simulink model "encelado"  (R2022b)
settings: Solver=ode4  StartTime=0.0  StopTime=500  FixedStep=0.01  RelTol=1e-3
values from neighbouring files (symbols this model uses):
  ba0 = 1e-3*randn(3,1)    [enceladus.m]
  bg0 = deg2rad(10/3600)*randn(3,1)    [enceladus.m]
  dp_in = [-5;40;0]    [enceladus.m]
  dt_alt = 0.1    [enceladus.m]
  dt_cam = 1    [enceladus.m]
  dt_imu = 0.02    [enceladus.m]
  Frcs = 22    [enceladus.m]
  g0 = 9.80665    [enceladus.m]
  Gam = 0.005    [enceladus.m]
  hth = 0.5    [enceladus.m]
  Isp = 300    [enceladus.m]
  Isp_rcs = 290    [enceladus.m]
  k_c = 0.01    [enceladus.m]
  k_h = 0.005    [enceladus.m]
  kC = 1    [enceladus.m]
  kd = 2*zeta*wn*J    [enceladus.m]
  Km = 5    [enceladus.m]
  kp = 2*J*wn^2    [enceladus.m]
  kS = 1    [enceladus.m]
  kw = 1    [enceladus.m]
  L = (P-r_sito')*E    [enceladus.m]
  m_in = 1000    [enceladus.m]
  mu = 7.21e9    (= 7210000000)    [enceladus.m]
  n = sqrt(muS/a^3)    [enceladus.m]
  N_alt = round(dt_alt/dt_imu)    [enceladus.m]
  N_cam = round(dt_cam/dt_imu)    [enceladus.m]
  N_st = round(dt_st/dt_imu)    [enceladus.m]
  P0 = diag([sigma_p0^2*ones(1,3),sigma_v0^2*ones(1,3),sigma_b0^2*ones(1,3)])    [enceladus.m]
  p_in = (R+h0)*uf    [enceladus.m]
  Pa0 = blkdiag(sigma_th0^2*eye(3),sigma_bg0^2*eye(3))    [enceladus.m]
  pf = (R-0.5)*u_f    [enceladus.m]
  q_in = [1 0 0 0]'    [enceladus.m]
  R = 252.1e3    (= 252100)    [enceladus.m]
  r_off = [0;0;0]    [enceladus.m]
  sigma_a = 5e-4    (= 0.0005)    [enceladus.m]
  sigma_ba = 1e-6    (= 1e-06)    [enceladus.m]
  sigma_c0 = 0.5    [enceladus.m]
  sigma_h0 = 0.2    [enceladus.m]
  sigma_st = 5e-5    (= 5e-05)    [enceladus.m]
  sigma_u = 1e-8    (= 1e-08)    [enceladus.m]
  sigma_v = 1e-5    (= 1e-05)    [enceladus.m]
  taumax_rcs = 2*Frcs*L    (= 26.4)    [enceladus.m]
  tgo_min = 10    [enceladus.m]
  Tm = 0.4    [enceladus.m]
  Uoff = 0.05    [enceladus.m]
  Uon = 0.2    [enceladus.m]
  vf = [0;0;0]    [enceladus.m]
  w_in = [0 0 0]'    [enceladus.m]
  x0_hat = [p_in+sigma_p0*randn(3,1);dp_in+sigma_v0*randn(3,1);zeros(3,1)]    [enceladus.m]
  xa0 = [q_hat0;zeros(3,1)]    [enceladus.m]
undefined symbols (not defined in the file or in its folder): h_rw_in, hmax_rw, tau_rcs, taumax_rw
libraries: simulink x1
settings Model: Creator=lorenzocipolla  LastModifiedBy=lorenzocipolla

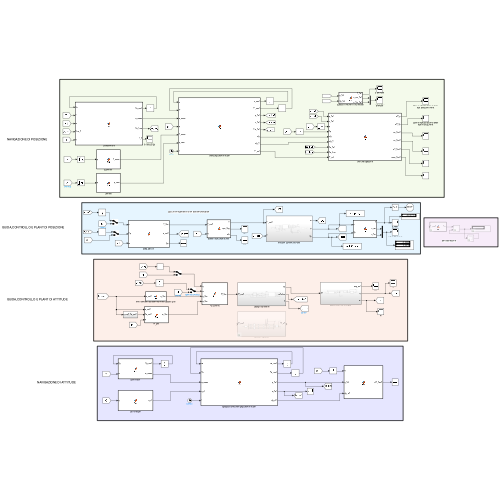
[thumbnail: Simulink's stored preview of the top-level diagram]
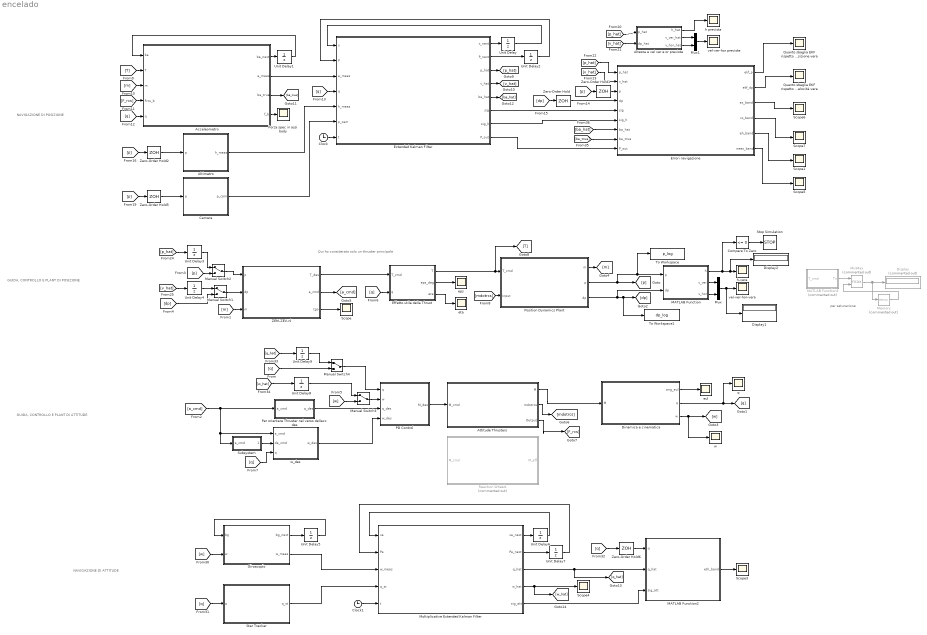
== system encelado ==
  note: NAVIGAZIONE DI POSIZIONE
  note: Qui ho considerato solo un thruster principale
  note: per saturazione
  note: GUIDA, CONTROLLO E PLANT DI POSIZIONE
  note: GUIDA, CONTROLLO E PLANT DI ATTITUDE
  note: NAVIGAZIONE DI ATTITUDE
  Acceleometro : MATLAB Function  TreatAsAtomicUnit=on
  Altezza e vel ver e or previste : MATLAB Function  TreatAsAtomicUnit=on
  Altimetro : MATLAB Function  TreatAsAtomicUnit=on
  Attitude Thrusters : Subsystem
  Camera : MATLAB Function  TreatAsAtomicUnit=on
  Clock : Clock
  Clock1 : Clock
  Compare To Zero : simulink/Logic and Bit Operations/Compare To Zero  relop=<=  OutDataTypeStr=boolean
  Dinamica e cinematica : Subsystem
  Display : Display  Commented=on
  Display1 : Display
  Display2 : Display
  Effetto utile della Thrust : MATLAB Function  TreatAsAtomicUnit=on
  Errori navigazione : MATLAB Function  TreatAsAtomicUnit=on
  Extended Kalman Filter : MATLAB Function  TreatAsAtomicUnit=on
  Forza spec in assi body : Scope
  Giroscopio : MATLAB Function  TreatAsAtomicUnit=on
  MATLAB Function : MATLAB Function  TreatAsAtomicUnit=on
  MATLAB Function2 : MATLAB Function  TreatAsAtomicUnit=on
  MATLAB Function3 : MATLAB Function  Commented=on  TreatAsAtomicUnit=on
  Manual Switch{1..4} (4 alike) : ManualSwitch
  Memory : Memory  Commented=on
  MinMax : MinMax  Commented=on  Function=max  Inputs=2
  Moltiplicative Extended Kalman Filter : MATLAB Function  TreatAsAtomicUnit=on
  Mux : Mux  Inputs=2
  Mux1 : Mux  Inputs=2
  PD Control : MATLAB Function  TreatAsAtomicUnit=on
  Per orientare Thruster nel verso dellacc des : MATLAB Function  TreatAsAtomicUnit=on
  Position Dynamics Plant : Subsystem
  Quanto sbaglia EKF rispetto alla posizione vera : Scope
  Quanto sbaglia EKF rispetto alla velocità vera : Scope
  Reaction Wheels : Subsystem  Commented=on
  Scope{,1,3..7} (7 alike) : Scope
  Star Tracker : MATLAB Function  TreatAsAtomicUnit=on
  Stop Simulation : Stop
  Subsystem : Subsystem
  To Workspace : ToWorkspace  VariableName=p_log  SampleTime=-1
  To Workspace1 : ToWorkspace  VariableName=dp_log  SampleTime=-1
  Unit Delay : UnitDelay  InitialCondition=x0_hat  SampleTime=dt_imu  HasFrameUpgradeWarning=on
  Unit Delay1 : UnitDelay  InitialCondition=ba0  SampleTime=dt_imu  HasFrameUpgradeWarning=on
  Unit Delay2 : UnitDelay  InitialCondition=P0  SampleTime=dt_imu  HasFrameUpgradeWarning=on
  Unit Delay3 : UnitDelay  InitialCondition=x0_hat(1:3)  SampleTime=dt_imu  HasFrameUpgradeWarning=on
  Unit Delay4 : UnitDelay  InitialCondition=x0_hat(4:6)  SampleTime=dt_imu  HasFrameUpgradeWarning=on
  Unit Delay5 : UnitDelay  InitialCondition=bg0  SampleTime=dt_imu  HasFrameUpgradeWarning=on
  Unit Delay6 : UnitDelay  InitialCondition=xa0  SampleTime=dt_imu  HasFrameUpgradeWarning=on
  Unit Delay7 : UnitDelay  InitialCondition=Pa0  SampleTime=dt_imu  HasFrameUpgradeWarning=on
  Unit Delay8 : UnitDelay  InitialCondition=xa0(5:7)  SampleTime=dt_imu  HasFrameUpgradeWarning=on
  Unit Delay9 : UnitDelay  InitialCondition=xa0(1:4)  SampleTime=dt_imu  HasFrameUpgradeWarning=on
  ZEM-ZEV-nl : MATLAB Function  TreatAsAtomicUnit=on
  Zero-Order Hold : ZeroOrderHold  SampleTime=dt_imu
  Zero-Order Hold1 : ZeroOrderHold  SampleTime=dt_imu
  Zero-Order Hold2 : ZeroOrderHold  SampleTime=dt_alt
  Zero-Order Hold5 : ZeroOrderHold  SampleTime=dt_cam
  Zero-Order Hold6 : ZeroOrderHold  SampleTime=dt_imu
  eps : Scope
  eta : Scope
  eul : Scope
  h prevista : Scope
  h-vera : Scope
  q : Scope
  vel-ver-hor previste : Scope
  vel-ver-hor-vera : Scope
  w : Scope
  w_des : MATLAB Function  TreatAsAtomicUnit=on
  wires:
  MinMax/1 -> Memory/1, Display/1
  Memory/1 -> MinMax/2
  MATLAB Function3/1(Tn) -> MinMax/1
  Dinamica e cinematica/1(ang_eul) -> eul/1
  Dinamica e cinematica/2(q) -> q/1, [q]
  Dinamica e cinematica/3(w) -> [w], w/1
  Position Dynamics Plant/2(p) -> To Workspace/1, MATLAB Function/1(p), [p]
  Position Dynamics Plant/3(dp) -> MATLAB Function/2(dp), To Workspace1/1, [dp]
  Position Dynamics Plant/1(m) -> [m]
  MATLAB Function/1(h) -> Display2/1, h-vera/1, Compare To Zero/1
  MATLAB Function/2(v_ver) -> Mux/1
  MATLAB Function/3(v_hor) -> Mux/2
  Mux/1 -> vel-ver-hor-vera/1, Display1/1
  [m] -> ZEM-ZEV-nl/3(m)
  ZEM-ZEV-nl/2(a_cmd) -> [a_cmd]
  [q] -> Effetto utile della Thrust/2(q)
  Effetto utile della Thrust/1(T) -> [T], Position Dynamics Plant/1(T_cmd)
  Effetto utile della Thrust/3(eta) -> eta/1
  Effetto utile della Thrust/2(eps_deg) -> eps/1
  ZEM-ZEV-nl/1(T_des) -> Effetto utile della Thrust/1(T_cmd)
  Compare To Zero/1 -> Stop Simulation/1
  ZEM-ZEV-nl/3(tgo) -> Scope/1
  Per orientare Thruster nel verso dellacc des/1(q_des) -> PD Control/3(q_des)
  w_des/1(w_des) -> PD Control/4(w_des)
  [a_cmd] -> Subsystem/1(a_cmd), w_des/1(a_cmd), Per orientare Thruster nel verso dellacc des/1(a_cmd)
  Subsystem/1(da_cmd) -> w_des/2(da_cmd)
  [q] -> w_des/3(q)
  PD Control/1(M_des) -> Attitude Thrusters/1(M_cmd)
  Attitude Thrusters/1(M) -> Dinamica e cinematica/1(M)
  [mdotrcs] -> Position Dynamics Plant/2(Input)
  Attitude Thrusters/2(mdotrcs) -> [mdotrcs]
  [T] -> Acceleometro/2(T)
  Attitude Thrusters/3(Output) -> [F_rcs]
  [F_rcs] -> Acceleometro/4(Frcs_b)
  [m] -> Acceleometro/3(m)
  [q] -> Acceleometro/5(q)
  Extended Kalman Filter/1(x_next) -> Unit Delay/1
  Unit Delay/1 -> Extended Kalman Filter/1(x)
  Acceleometro/1(ba_next) -> Unit Delay1/1
  Unit Delay1/1 -> Acceleometro/1(ba)
  Acceleometro/2(a_meas) -> Extended Kalman Filter/3(a_meas)
  [q] -> Extended Kalman Filter/4(q)
  Acceleometro/4(f_b) -> Forza spec in assi body/1
  Altezza e vel ver e or previste/3(v_hor_hat) -> Mux1/2
  Altezza e vel ver e or previste/2(v_ver_hat) -> Mux1/1
  Altezza e vel ver e or previste/1(h_hat) -> h prevista/1
  Mux1/1 -> vel-ver-hor previste/1
  Errori navigazione/1(ekf_p) -> Quanto sbaglia EKF rispetto alla posizione vera/1
  Errori navigazione/2(ekf_dp) -> Quanto sbaglia EKF rispetto alla velocità vera/1
  [p] -> Zero-Order Hold1/1
  Zero-Order Hold1/1 -> Errori navigazione/3(p)
  Zero-Order Hold/1 -> Errori navigazione/4(dp)
  [dp] -> Zero-Order Hold/1
  Errori navigazione/3(ex_band) -> Scope6/1
  Errori navigazione/4(vx_band) -> Scope7/1
  Extended Kalman Filter/2(P_next) -> Unit Delay2/1
  Unit Delay2/1 -> Extended Kalman Filter/2(P)
  Extended Kalman Filter/6(sig) -> Errori navigazione/5(sig)
  [p] -> Zero-Order Hold2/1
  Zero-Order Hold2/1 -> Altimetro/1(p)
  Clock/1 -> Extended Kalman Filter/7(t)
  Altimetro/1(h_meas) -> Extended Kalman Filter/5(h_meas)
  Extended Kalman Filter/7(sig_h) -> Errori navigazione/6(sig_h)
  Errori navigazione/5(eh_band) -> Scope1/1
  Camera/1(p_cam) -> Extended Kalman Filter/6(p_cam)
  [p] -> Zero-Order Hold5/1
  Zero-Order Hold5/1 -> Camera/1(p)
  Extended Kalman Filter/4(v_hat) -> [v_hat]
  Extended Kalman Filter/3(p_hat) -> [p_hat]
  [p_hat] -> Altezza e vel ver e or previste/1(p_hat)
  [v_hat] -> Altezza e vel ver e or previste/2(dp_hat)
  [p_hat] -> Errori navigazione/1(p_hat)
  [v_hat] -> Errori navigazione/2(v_hat)
  Acceleometro/3(ba_true) -> [ba_true]
  Extended Kalman Filter/5(ba_hat) -> [ba_hat]
  [p_hat] -> Unit Delay3/1
  [v_hat] -> Unit Delay4/1
  Manual Switch1/1 -> ZEM-ZEV-nl/2(dp)
  Manual Switch2/1 -> ZEM-ZEV-nl/1(p)
  [p] -> Manual Switch2/2
  Unit Delay3/1 -> Manual Switch2/1
  Unit Delay4/1 -> Manual Switch1/1
  [dp] -> Manual Switch1/2
  [w] -> Giroscopio/2(w)
  Giroscopio/1(bg_next) -> Unit Delay5/1
  Unit Delay5/1 -> Giroscopio/1(bg)
  [q] -> Star Tracker/1(q)
  Moltiplicative Extended Kalman Filter/1(xa_next) -> Unit Delay6/1
  Unit Delay6/1 -> Moltiplicative Extended Kalman Filter/1(xa)
  Giroscopio/2(w_meas) -> Moltiplicative Extended Kalman Filter/3(w_meas)
  Moltiplicative Extended Kalman Filter/3(q_hat) -> [q_hat], MATLAB Function2/2(q_hat)
  Moltiplicative Extended Kalman Filter/5(sig_att) -> MATLAB Function2/3(sig_att)
  MATLAB Function2/1(eth_band) -> Scope3/1
  Moltiplicative Extended Kalman Filter/2(Pa_next) -> Unit Delay7/1
  Unit Delay7/1 -> Moltiplicative Extended Kalman Filter/2(Pa)
  Star Tracker/1(q_st) -> Moltiplicative Extended Kalman Filter/4(q_st)
  Zero-Order Hold6/1 -> MATLAB Function2/1(q)
  [q] -> Zero-Order Hold6/1
  Clock1/1 -> Moltiplicative Extended Kalman Filter/5(t)
  Moltiplicative Extended Kalman Filter/4(w_hat) -> [w_hat], Scope4/1
  [q_hat] -> Unit Delay9/1
  [w_hat] -> Unit Delay8/1
  Manual Switch3/1 -> PD Control/2(w)
  [w] -> Manual Switch3/2
  Unit Delay8/1 -> Manual Switch3/1
  [q] -> Manual Switch4/2
  Unit Delay9/1 -> Manual Switch4/1
  Manual Switch4/1 -> PD Control/1(q)
  Errori navigazione/6(nees_band) -> Scope5/1
  [ba_true] -> Errori navigazione/8(ba_true)
  [ba_hat] -> Errori navigazione/7(ba_hat)
  Extended Kalman Filter/8(P_out) -> Errori navigazione/9(P_out)

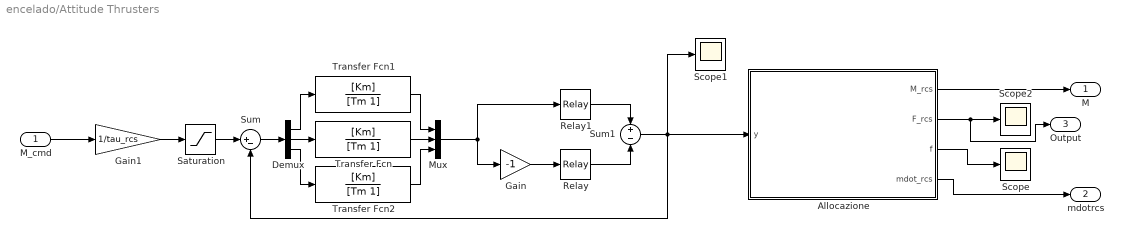
== system encelado/Attitude Thrusters ==
  M_cmd : Inport
  Allocazione : MATLAB Function  TreatAsAtomicUnit=on
  Demux : Demux  Outputs=3
  Gain : Gain  Gain=-1
  Gain1 : Gain  Gain=1/tau_rcs
  Mux : Mux  Inputs=3
  Relay : Relay  OnSwitchValue=Uon  OffSwitchValue=Uoff
  Relay1 : Relay  OnSwitchValue=Uon  OffSwitchValue=Uoff
  Saturation : Saturate  UpperLimit=taumax_rcs  LowerLimit=-taumax_rcs
  Scope : Scope
  Scope1 : Scope
  Scope2 : Scope
  Sum : Sum  Inputs=|+-
  Sum1 : Sum  Inputs=+|-
  Transfer Fcn : TransferFcn  Numerator=[Km]  Denominator=[Tm 1]
  Transfer Fcn1 : TransferFcn  Numerator=[Km]  Denominator=[Tm 1]
  Transfer Fcn2 : TransferFcn  Numerator=[Km]  Denominator=[Tm 1]
  M : Outport
  mdotrcs : Outport  Port=2
  Output : Outport  Port=3
  wires:
  Gain/1 -> Relay/1
  Sum1/1 -> Allocazione/1(y), Sum/2, Scope1/1
  Saturation/1 -> Sum/1
  Relay/1 -> Sum1/2
  Relay1/1 -> Sum1/1
  Gain1/1 -> Saturation/1
  Sum/1 -> Demux/1
  Demux/2 -> Transfer Fcn/1
  Transfer Fcn/1 -> Mux/2
  Demux/1 -> Transfer Fcn1/1
  Demux/3 -> Transfer Fcn2/1
  Transfer Fcn1/1 -> Mux/1
  Transfer Fcn2/1 -> Mux/3
  Mux/1 -> Gain/1, Relay1/1
  Allocazione/4(mdot_rcs) -> mdotrcs/1
  Allocazione/2(F_rcs) -> Output/1, Scope2/1
  Allocazione/3(f) -> Scope/1
  Allocazione/1(M_rcs) -> M/1
  M_cmd/1 -> Gain1/1

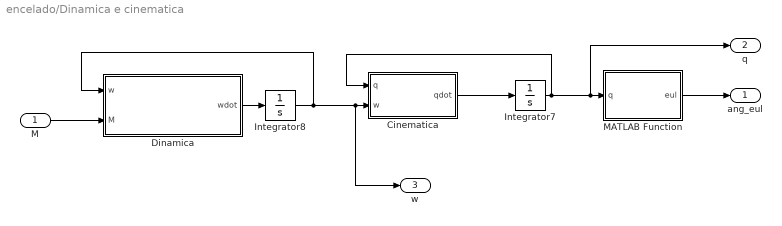
== system encelado/Dinamica e cinematica ==
  M : Inport
  Cinematica : MATLAB Function  TreatAsAtomicUnit=on
  Dinamica : MATLAB Function  TreatAsAtomicUnit=on
  Integrator7 : Integrator  InitialCondition=q_in
  Integrator8 : Integrator  InitialCondition=w_in
  MATLAB Function : MATLAB Function  TreatAsAtomicUnit=on
  ang_eul : Outport
  q : Outport  Port=2
  w : Outport  Port=3
  wires:
  Integrator7/1 -> q/1, MATLAB Function/1(q), Cinematica/1(q)
  Cinematica/1(qdot) -> Integrator7/1
  Dinamica/1(wdot) -> Integrator8/1
  MATLAB Function/1(eul) -> ang_eul/1
  Integrator8/1 -> Dinamica/1(w), w/1, Cinematica/2(w)
  M/1 -> Dinamica/2(M)

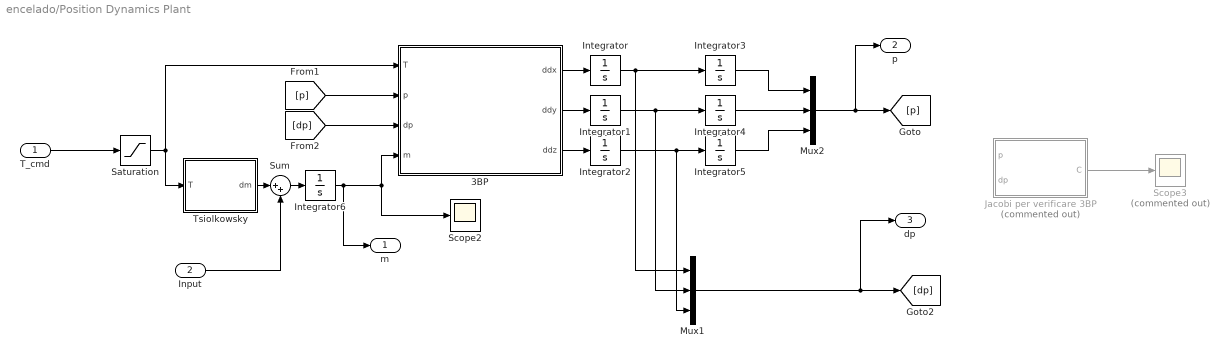
== system encelado/Position Dynamics Plant ==
  T_cmd : Inport
  Input : Inport  Port=2
  3BP : MATLAB Function  TreatAsAtomicUnit=on
  Integrator : Integrator  InitialCondition=dp_in(1)
  Integrator1 : Integrator  InitialCondition=dp_in(2)
  Integrator2 : Integrator  InitialCondition=dp_in(3)
  Integrator3 : Integrator  InitialCondition=p_in(1)
  Integrator4 : Integrator  InitialCondition=p_in(2)
  Integrator5 : Integrator  InitialCondition=p_in(3)
  Integrator6 : Integrator  InitialCondition=m_in
  Jacobi per verificare 3BP : MATLAB Function  Commented=on  TreatAsAtomicUnit=on
  Mux1 : Mux  Inputs=3
  Mux2 : Mux  Inputs=3
  Saturation : Saturate  UpperLimit=700  LowerLimit=-700
  Scope2 : Scope
  Scope3 : Scope  Commented=on
  Sum : Sum  Inputs=|++
  Tsiolkowsky : MATLAB Function  TreatAsAtomicUnit=on
  m : Outport
  p : Outport  Port=2
  dp : Outport  Port=3
  wires:
  3BP/3(ddz) -> Integrator2/1
  Integrator4/1 -> Mux2/2
  Mux1/1 -> dp/1, [dp]
  3BP/1(ddx) -> Integrator/1
  Integrator5/1 -> Mux2/3
  Mux2/1 -> p/1, [p]
  Integrator6/1 -> Scope2/1, 3BP/4(m), m/1
  Integrator2/1 -> Integrator5/1, Mux1/3
  Integrator/1 -> Mux1/1, Integrator3/1
  Saturation/1 -> 3BP/1(T), Tsiolkowsky/1(T)
  Integrator3/1 -> Mux2/1
  Integrator1/1 -> Mux1/2, Integrator4/1
  T_cmd/1 -> Saturation/1
  3BP/2(ddy) -> Integrator1/1
  [p] -> 3BP/2(p)
  [dp] -> 3BP/3(dp)
  Jacobi per verificare 3BP/1(C) -> Scope3/1
  Tsiolkowsky/1(dm) -> Sum/1
  Sum/1 -> Integrator6/1
  Input/1 -> Sum/2

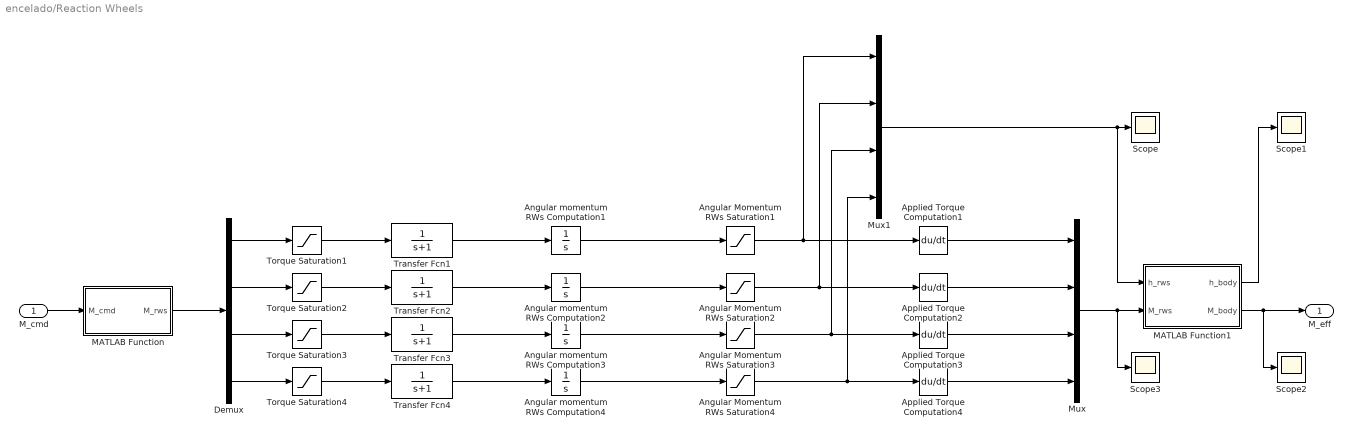
== system encelado/Reaction Wheels ==
  M_cmd : Inport
  Angular Momentum RWs Saturation{1..4} (4 alike) : Saturate  UpperLimit=hmax_rw  LowerLimit=-hmax_rw
  Angular momentum RWs Computation1 : Integrator  InitialCondition=h_rw_in(1)
  Angular momentum RWs Computation2 : Integrator  InitialCondition=h_rw_in(2)
  Angular momentum RWs Computation3 : Integrator  InitialCondition=h_rw_in(3)
  Angular momentum RWs Computation4 : Integrator  InitialCondition=h_rw_in(4)
  Applied Torque Computation{1..4} (4 alike) : Derivative  CoefficientInTFapproximation=0.01
  Demux : Demux
  MATLAB Function : MATLAB Function  TreatAsAtomicUnit=on
  MATLAB Function1 : MATLAB Function  TreatAsAtomicUnit=on
  Mux : Mux
  Mux1 : Mux
  Scope{,1..3} (4 alike) : Scope
  Torque Saturation{1..4} (4 alike) : Saturate  UpperLimit=taumax_rw  LowerLimit=-taumax_rw
  Transfer Fcn{1..4} (4 alike) : TransferFcn  Denominator=[1 1]
  M_eff : Outport
  wires:
  M_cmd/1 -> MATLAB Function/1(M_cmd)
  MATLAB Function/1(M_rws) -> Demux/1
  Torque Saturation1/1 -> Transfer Fcn1/1
  Transfer Fcn2/1 -> Angular momentum RWs Computation2/1
  Demux/2 -> Torque Saturation2/1
  Angular Momentum RWs Saturation3/1 -> Mux1/3, Applied Torque Computation3/1
  Torque Saturation4/1 -> Transfer Fcn4/1
  Torque Saturation2/1 -> Transfer Fcn2/1
  Angular momentum RWs Computation2/1 -> Angular Momentum RWs Saturation2/1
  Transfer Fcn4/1 -> Angular momentum RWs Computation4/1
  Angular Momentum RWs Saturation1/1 -> Mux1/1, Applied Torque Computation1/1
  Applied Torque Computation4/1 -> Mux/4
  Angular momentum RWs Computation3/1 -> Angular Momentum RWs Saturation3/1
  Torque Saturation3/1 -> Transfer Fcn3/1
  Angular Momentum RWs Saturation2/1 -> Mux1/2, Applied Torque Computation2/1
  Applied Torque Computation3/1 -> Mux/3
  Angular momentum RWs Computation4/1 -> Angular Momentum RWs Saturation4/1
  Demux/1 -> Torque Saturation1/1
  Applied Torque Computation2/1 -> Mux/2
  Applied Torque Computation1/1 -> Mux/1
  Transfer Fcn3/1 -> Angular momentum RWs Computation3/1
  Angular momentum RWs Computation1/1 -> Angular Momentum RWs Saturation1/1
  Demux/3 -> Torque Saturation3/1
  Transfer Fcn1/1 -> Angular momentum RWs Computation1/1
  Angular Momentum RWs Saturation4/1 -> Mux1/4, Applied Torque Computation4/1
  Demux/4 -> Torque Saturation4/1
  MATLAB Function1/2(M_body) -> Scope2/1, M_eff/1
  Mux/1 -> Scope3/1, MATLAB Function1/2(M_rws)
  Mux1/1 -> MATLAB Function1/1(h_rws), Scope/1
  MATLAB Function1/1(h_body) -> Scope1/1

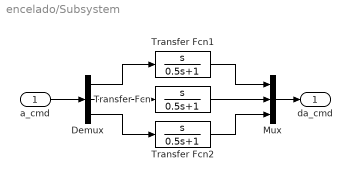
== system encelado/Subsystem ==
  a_cmd : Inport
  Demux : Demux  Outputs=3
  Mux : Mux  Inputs=3
  Transfer Fcn : TransferFcn  Numerator=[1 0]  Denominator=[0.5 1]
  Transfer Fcn1 : TransferFcn  Numerator=[1 0]  Denominator=[0.5 1]
  Transfer Fcn2 : TransferFcn  Numerator=[1 0]  Denominator=[0.5 1]
  da_cmd : Outport
  wires:
  Transfer Fcn2/1 -> Mux/3
  Demux/2 -> Transfer Fcn/1
  Demux/1 -> Transfer Fcn1/1
  Transfer Fcn1/1 -> Mux/1
  a_cmd/1 -> Demux/1
  Demux/3 -> Transfer Fcn2/1
  Transfer Fcn/1 -> Mux/2
  Mux/1 -> da_cmd/1

== matlab function encelado/MATLAB Function3 ==
  data: T_cmd input; Tn output
function Tn = fcn(T_cmd)
Tn=norm(T_cmd);

== matlab function encelado/Dinamica e cinematica/Cinematica ==
  data: q input; qdot output; w input
function qdot = fcn(q,w)
wx=w(1); wy=w(2); wz=w(3);
OM=[0  -wx -wy -wz;
    wx  0   wz -wy;
    wy -wz  0   wx;
    wz  wy  -wx  0];

qdot=1/2*OM*q;

== matlab function encelado/Dinamica e cinematica/Dinamica ==
  data: wdot output; w input; J parameter; M input
function wdot=fcn(w,J,M)
h=J*w;
cro=cross(w,h);
wdot=J\(M-cro); %è la stessa cosa di dire invJ) ma è più robusto

== matlab function encelado/Dinamica e cinematica/MATLAB Function ==
  data: q input; eul output
function eul=fcn(q)
q=q(:)/norm(q);
phi=atan2(2*(q(3)*q(4)+q(1)*q(2)),1-2*(q(2)^2+q(3)^2));
theta=-asin(max(-1,min(1,2*(q(2)*q(4)-q(1)*q(3)))));
psi=atan2(2*(q(2)*q(3)+q(1)*q(4)),1-2*(q(3)^2+q(4)^2));
eul=[phi theta psi]';

== matlab function encelado/Reaction Wheels/MATLAB Function ==
  data: M_cmd input; M_rws output; Z parameter
function M_rws = fcn(M_cmd,Z)
M_rws=pinv(Z)*M_cmd

== matlab function encelado/Reaction Wheels/MATLAB Function1 ==
  data: h_body output; h_rws input; M_body output; M_rws input; Z parameter
function [h_body, M_body]= fcn(h_rws,M_rws,Z)

h_body=Z*h_rws;
M_body=Z*M_rws;

== matlab function encelado/PD Control ==
  data: q input size=4; M_des output size=3; w input size=3; kp parameter; kd parameter; q_des input size=4; w_des input size=3
function M_des=fcn(q,w,kp, kd, q_des, w_des)
qr=q(:)'/norm(q); 
qdr=q_des(:)'/norm(q_des);
%forza il vettore da colonna a riga, normq serve per non farlo impazzire, 
%ci serve perche qinv qmultiply lavorano su vettori riga, poi nel pd li
%trasformo di nuovo in colonna
deq=quatmultiply(quatinv(qr),qdr);
dq0=deq(1);        %tanto è scalare
deqvec=deq(2:4)';  %ritrasformo in colonna
M_des=kp*sign(dq0)*deqvec+kd*(w_des-w);

== matlab function encelado/Per orientare Thruster nel verso dellacc des ==
  data: a_cmd input size=3; q_des output size=4
function q_des=fcn(a_cmd)

if norm(a_cmd)<1e-9
    q_des=[1;0;0;0];
    return
end

a_cmd=a_cmd(:)/norm(a_cmd); %forza a_cmd ad essere colonna, anche se già 
%lo era ma lo metto per ridondanza e lo normalizza, diventa un versore
b0=[0 0 1]';
c=dot(a_cmd,b0);
if c>0.9999
    q_des=[1 0 0 0]';
elseif c<-0.9999
    q_des=[0 1 0 0]';
else
    e=cross(b0,a_cmd);
    e_cap=e/norm(e);
    theta=acos(max(-1,min(1,c)));
    q_des=[cos(theta/2);e_cap*sin(theta/2)];
end

== matlab function encelado/Effetto utile della Thrust ==
  data: T_cmd input size=3; T output size=3; q input size=4; eps_deg output; eta output
function [T,eps_deg,eta]=fcn(T_cmd,q)
q=q(:)/norm(q);
qs=q(1); qv=q(2:4);
A=(qs^2-qv'*qv)*eye(3)+2*(qv*qv')-2*qs*[0 -qv(3) qv(2);qv(3) 0 -qv(1);-qv(2) qv(1) 0];
b0=[0;0;1];
b_cap=A'*b0; %trasposta: da SR body a SR inerziale
Tn=max(0,dot(T_cmd,b_cap)); %spinta non negativa, il motore spinge e non tira
T=Tn*b_cap;

%Errore di puntamento
nT=norm(T_cmd);
if nT<1e-9
    eps_deg=0; eta=1; %spinta nulla (cutoff): errore non definito
else
    c=max(-1,min(1,dot(b_cap,T_cmd/nT)));
    eps_deg=acosd(c); %angolo tra asse motore e direzione comandata [deg]
    eta=max(0,c);     %frazione della spinta comandata realmente erogata
end

== matlab function encelado/w_des ==
  data: a_cmd input size=3; w_des output size=3; da_cmd input size=3; q input size=4
function w_des=fcn(a_cmd,da_cmd,q)
na=norm(a_cmd);
if na<1e-9
    w_des=zeros(3,1);
    return
end
q=q(:)/norm(q);
qs=q(1); qv=q(2:4);
A=(qs^2-qv'*qv)*eye(3)+2*(qv*qv')-2*qs*[0 -qv(3) qv(2);qv(3) 0 -qv(1);-qv(2) qv(1) 0];
ah=a_cmd/na;
acapdot=(da_cmd-ah*(ah'*da_cmd))/na;
w_des=A*cross(ah,acapdot);

== matlab function encelado/Attitude Thrusters/Allocazione ==
  data: y input; M_rcs output; F_rcs output; f output; mdot_rcs output; Frcs parameter; Isp_rcs parameter; L parameter; hth parameter; r_off parameter; g0 parameter
function [M_rcs,F_rcs,f,mdot_rcs]=fcn(y,Frcs, Isp_rcs, L, hth, r_off, g0)
%Propulsori di assetto (RCS): 12 propulsori, 4 grappoli sugli spigoli superiori
%colonne 1-2:+x  3-4:-x  5-6:+y  7-8:-y  9-10:+z  11-12:-z
Rth=[0 0 0 0 L -L L -L L -L 0 0;
     -L L -L L 0 0 0 0 0 0 L -L;
     hth*ones(1,12)];
Dth=[0 0 0 0 0 0 0 0 0 0 1 -1;
     0 0 0 0 0 0 0 0 1 -1 0 0;
     -1 1 1 -1 -1 1 1 -1 0 0 0 0];
Bm=zeros(3,12);
for k=1:12
    Bm(:,k)=Frcs*cross(Rth(:,k)-r_off,Dth(:,k));
end
Fm=Frcs*Dth;
%Allocazione: quali propulsori accendere per il comando y (+1/0/-1)
f=zeros(12,1);
if y(1)>0.5
    f(1:2)=1;            %coppia +x
elseif y(1)<-0.5
    f(3:4)=1;            %coppia -x
end
if y(2)>0.5
    f(5:6)=1;            %coppia +y
elseif y(2)<-0.5
    f(7:8)=1;            %coppia -y
end
if y(3)>0.5
    f(9:10)=1;           %coppia +z
elseif y(3)<-0.5
    f(11:12)=1;          %coppia -z
end
M_rcs=Bm*f;                          %coppia totale [N m]
F_rcs=Fm*f;                          %forza netta [N]
mdot_rcs=-Frcs*sum(f)/(Isp_rcs*g0);  %consumo [kg/s]

== matlab function encelado/Acceleometro ==
  settings: updateMethod=DISCRETE  sampleTime=dt_imu
  data: ba input; ba_next output; a_meas output; T input; m input; Frcs_b input; q input; ba_true output; f_b output; sigma_a parameter; dt_imu parameter; sigma_ba parameter
function [ba_next,a_meas,ba_true,f_b]=fcn(ba,T,m,Frcs_b,q,sigma_a,dt_imu,sigma_ba)

%Simula un accelerometro montato sul lander: prende lo stato vero dal plant e restituisce cio' che il sensore leggerebbe davvero, 
%cioe' il valore vero rovinato dai difetti del sensore (rumore bianco + bias con random walk).
%Serve perche' il computer di bordo non conosce p e dp veri: li deve stimare.
%Il filtro integra queste misure per ricostruire velocita' e posizione (step 2),poi altimetro e camera correggono la deriva (step 4-5).
%L'accelerometro misura la forza specifica: non vede gravita' ne' termini di Hill, perche' g agisce allo stesso modo sulla massa di prova 
% e sul satellite.
% Il bias e' uno stato: lo ricorda il Unit Delay esterno (IC=ba0, Ts=dt_imu).

%ROTAZIONE HILL -> CORPO
%L'accelerometro e' fissato al lander, quindi misura in assi corpo: serve la matrice che porta i vettori dal frame di Hill a quello body.
q=q(:)/norm(q); qs=q(1); qv=q(2:4);   %quaternione normalizzato, parte scalare e vettoriale
A=(qs^2-qv'*qv)*eye(3)+2*(qv*qv')-2*qs*[0 -qv(3) qv(2);qv(3) 0 -qv(1);-qv(2) qv(1) 0]; %matrice Hill -> corpo

%FORZA SPECIFICA VERA
%Solo le forze non gravitazionali (spinta principale + RCS) divise per la massa.
f_b=A*T/m+Frcs_b/m;                   %T e' in Hill (va ruotata), Frcs_b e' gia' in corpo

%MISURA CON I DIFETTI DEL SENSORE
%Alla forza specifica vera si aggiungono il bias del passo corrente e il rumore bianco.
nk=randn(3,1);                        %campione gaussiano standard
eta_a=(sigma_a/sqrt(dt_imu))*nk;      %rumore bianco discreto a media nulla (densita' sigma_a -> varianza sigma_a^2/dt)
a_meas=f_b+ba+eta_a;                  %misura dell'accelerometro
ba_true=ba;                           %bias vero usato in questa misura (per confrontarlo con ba_hat)

%EVOLUZIONE DEL BIAS
%Il bias deriva lentamente (random walk). Il valore calcolato qui torna in ingresso al passo successivo tramite il Unit Delay.
wk=randn(3,1);                        %campione gaussiano standard
ba_next=ba+sigma_ba*sqrt(dt_imu)*wk;  %bias al passo successivo

== matlab function encelado/Extended Kalman Filter ==
  settings: updateMethod=DISCRETE  sampleTime=dt_imu
  data: x input; P input; x_next output size=9; P_next output; p_hat output size=3; v_hat output size=3; a_meas input; q input; h_meas input; p_cam input; t input; n parameter; kC parameter; ba_hat output size=3; kS parameter; kw parameter; mu parameter; dt_imu parameter; sig output; sig_h output; sigma_a parameter; sigma_ba parameter; k_h parameter; R parameter; sigma_h0 parameter; N_alt parameter; sigma_c0 parameter; N_cam parameter; k_c parameter; P_out output
function [x_next,P_next,p_hat,v_hat,ba_hat,sig,sig_h,P_out]=fcn(x,P,a_meas,q,h_meas,p_cam,t,n,kC,kS,kw,mu,dt_imu,sigma_a,sigma_ba,k_h,R,sigma_h0,N_alt,sigma_c0, N_cam, k_c)

%EKF di navigazione. Stato x=[p;v;ba] (9x1) nel frame di Hill.
%A ogni passo: 1) corregge con l'altimetro se c'e' una misura nuova, 2) calcola le uscite, 3) propaga stato e covarianza al passo successivo.

%CORREZIONE CON L'ALTIMETRO
%Solo ai passi in cui arriva una misura nuova (ogni N_alt passi IMU):confronta la quota misurata con quella prevista e aggiorna x e P.
y_h=0; sS_h=0;                        %innovazione e sua sigma (0 se non c'e' misura)
k=round(t/dt_imu);                    %indice del passo IMU corrente
if mod(k,N_alt)==0                    %vero solo quando arriva una misura dell'altimetro
    p=x(1:3); r=norm(p); u=p/r;       %posizione prevista, distanza dal centro, versore radiale
    h_hat=r-R;                        %quota prevista
    sigma_h=sigma_h0+k_h*max(h_hat,0);%rumore dell'altimetro alla quota prevista
    H=[u' zeros(1,6)];                %jacobiano dh/dx: la quota dipende solo da p, lungo u
    y_h=h_meas-h_hat;                 %innovazione: misura - previsione
    S=H*P*H'+sigma_h^2;               %varianza dell'innovazione (previsione + sensore)
    K=P*H'/S;                         %guadagno 9x1: quanto correggere ogni componente
    x=x+K*y_h;                        %stato corretto
    IKH=eye(9)-K*H;
    P=IKH*P*IKH'+K*sigma_h^2*K';      %covarianza corretta (forma di Joseph, resta simmetrica e positiva)
    sS_h=sqrt(max(S,0));              %sigma dell'innovazione, per il test y_h entro +-3sS_h
    dbg=[S;norm(x);norm(q);min(real(eig(0.5*(P+P'))))]; %S, norma stato, norma quaternione, autovalore minimo di P
end

%CORREZIONE CON LA CAMERA
%Solo ai passi in cui arriva un fix della camera (ogni N_cam passi IMU):
%confronta la posizione misurata con quella prevista e aggiorna x e P.
%Stessa struttura dell'altimetro, ma la misura e' 3D e lineare nello stato.
if mod(k,N_cam)==0                    %vero solo quando arriva una misura della camera
    p=x(1:3);                         %posizione prevista (gia' corretta dall'altimetro se e' arrivato anche lui)
    h_hat=norm(p)-R;                  %quota stimata (serve solo per la sigma della camera)
    sigma_c=max(sigma_c0,k_c*h_hat);  %rumore atteso della camera alla quota stimata
    Hc=[eye(3) zeros(3,6)];           %la camera vede solo la posizione: niente jacobiano da calcolare
    Rc=sigma_c^2*eye(3);              %covarianza del rumore, uguale e indipendente sui tre assi
    y_c=p_cam(:)-p;                   %innovazione 3x1: misura - previsione
    Sc=Hc*P*Hc'+Rc;                   %covarianza dell'innovazione 3x3 (previsione + sensore)
    Kc=P*Hc'/Sc;                      %guadagno 9x3: quanto correggere ogni componente
    x=x+Kc*y_c;                       %stato corretto (anche v e bias, tramite le correlazioni in P)
    IKH=eye(9)-Kc*Hc;
    P=IKH*P*IKH'+Kc*Rc*Kc';           %covarianza corretta (forma di Joseph, resta simmetrica e positiva)
end

%USCITE AL PASSO k (dopo la correzione)
%Estrae la stima corrente e le deviazioni standard per i test +-3sigma.
p_hat=x(1:3); v_hat=x(4:6); ba_hat=x(7:9); %posizione, velocita', bias stimati
sig=sqrt(abs(diag(P)));               %sigma di ogni componente dello stato
uh=p_hat/norm(p_hat);                 %versore radiale stimato
sig_h=sqrt(abs(uh'*P(1:3,1:3)*uh));   %sigma della quota stimata (P di posizione proiettata sulla radiale)

%PROPAGAZIONE DELLO STATO (dalle eq della dinamica)
%Dead reckoning: accelerazione = modello (gravita' + Hill) + accelerometro riportato in Hill, poi integrazione su un passo dt_imu.
q=q(:)/norm(q); qs=q(1); qv=q(2:4); %quat normalizzato, parte scalare e vettoriale
A=(qs^2-qv'*qv)*eye(3)+2*(qv*qv')-2*qs*[0 -qv(3) qv(2);qv(3) 0 -qv(1);-qv(2) qv(1) 0]; %matrice Hill -> corpo
p=p_hat; v=v_hat; r=norm(p);
g=[ kC*2*n*v(2)+kw*n^2*p(1)+kS*2*n^2*p(1);
   -kC*2*n*v(1)+kw*n^2*p(2)-kS*n^2*p(2);
   -kS*n^2*p(3)]-mu*p/r^3;            %termini di Hill + gravita' di Encelado (non visti dall'accelerometro)
a_hat=g+A'*(a_meas-ba_hat);           %accelerazione totale stimata: modello + forza specifica senza bias, in Hill
x_next=x;                             %il bias resta costante nella previsione
x_next(1:3)=p+v*dt_imu+0.5*a_hat*dt_imu^2; %posizione al passo successivo
x_next(4:6)=v+a_hat*dt_imu;           %velocita' al passo successivo

%PROPAGAZIONE DELLA COVARIANZA
%Linearizza la dinamica (F), la discretizza (Phi) e fa crescere l'incertezza con il rumore dell'accelerometro e del bias (Qd).
u=p/r;                                %versore radiale
Gp=n^2*diag([kw+2*kS,kw-kS,-kS])-mu/r^3*(eye(3)-3*(u*u')); %d(accelerazione)/dp: Hill + gradiente di gravita'
Gv=2*n*kC*[0 1 0;-1 0 0;0 0 0];       %d(accelerazione)/dv: termine di Coriolis
F=zeros(9);                           %jacobiano della dinamica continua
F(1:3,4:6)=eye(3);                    %dp/dt=v
F(4:6,1:3)=Gp;
F(4:6,4:6)=Gv;
F(4:6,7:9)=-A';                       %il bias entra nell'accelerazione con segno meno
Phi=eye(9)+F*dt_imu+0.5*(F*F)*dt_imu^2; %matrice di transizione discreta (Taylor 2o ordine)
Qd=zeros(9);                          %rumore di processo discreto
Qd(4:6,4:6)=sigma_a^2*dt_imu*eye(3);  %rumore accelerometro -> incertezza sulla velocita'
Qd(7:9,7:9)=sigma_ba^2*dt_imu*eye(3); %random walk del bias
P_next=Phi*P*Phi'+Qd;                 %covarianza al passo successivo
P_next=0.5*(P_next+P_next');          %forza la simmetria (elimina errori numerici)
P_out=P;

== matlab function encelado/Altezza e vel ver e or previste ==
  data: p_hat input size=3; dp_hat input size=3; R parameter; h_hat output size=1; v_ver_hat output; v_hor_hat output
function [h_hat,v_ver_hat,v_hor_hat]=fcn(p_hat,dp_hat,R)
u_hat=p_hat/norm(p_hat);
h_hat=norm(p_hat)-R;
v_ver_hat=dp_hat'*u_hat;
v_hor_hat=norm(dp_hat-v_ver_hat*u_hat);

== matlab function encelado/Errori navigazione ==
  data: p_hat input; v_hat input; p input; ekf_p output; dp input; ekf_dp output; sig input; ex_band output; vx_band output; eh_band output; R parameter; sig_h input; nees_band output; ba_hat input; ba_true input; P_out input
function [ekf_p,ekf_dp,ex_band,vx_band,eh_band,nees_band]=fcn(p_hat,v_hat,p,dp,sig,R,sig_h,ba_hat,ba_true,P_out)
%Errori di navigazione: confronta la stima del filtro con lo stato vero (noto solo in simulazione) per valutare se l'EKF funziona.
%p e dp arrivano dal plant tramite Zero-Order Hold con dt_imu, cosi' sono
%campionati allo stesso istante della stima (niente banda di sfasamento).
%Blocco senza stato: non serve nessun Unit Delay.

%MODULI DEGLI ERRORI
%Quanto e' lontana la stima dalla verita', in totale.
ekf_p=norm(p_hat-p);                  %modulo errore di posizione [m]
ekf_dp=norm(v_hat-dp);                %modulo errore di velocita' [m/s]

%TEST +-3SIGMA SULLA COMPONENTE X
%Vettore [errore vero; +3sigma; -3sigma] da mandare a uno Scope: se il filtro e'coerente l'errore resta dentro la banda. x e' quasi la verticale.
ex_band=[p_hat(1)-p(1);3*sig(1);-3*sig(1)]; %posizione x: sig(1)=sigma di p_x
vx_band=[v_hat(1)-dp(1);3*sig(4);-3*sig(4)]; %velocita' x: sig(4)=sigma di v_x

eh_band=[(norm(p_hat)-R)-(norm(p)-R);3*sig_h;-3*sig_h]; %errore di quota e banda +-3sigma

%======NEES BAND=====
%NEES (Normalized Estimation Error Squared): test di consistenza dell'EKF su tutto lo stato insieme, non componente per componente come il +-3sigma.
%Misura se l'errore vero e' grande quanto il filtro "crede" (P). p e v veri passati per Zero-Order Hold con dt_imu. Blocco senza stato.

%= ERRORE VERO ==========
x_hat=[p_hat;v_hat;ba_hat];           %stato stimato 9x1
x=[p;dp;ba_true];                      %stato vero 9x1 (noto solo in simulazione)
e=x_hat-x;                            %errore vero 9x1

% NEES E LIMITI ==========
%Se il filtro e' coerente il NEES segue una chi-quadro con 9 gradi di liberta':media 9, e il 95% dei campioni tra chi2inv(0.025,9) e chi2inv(0.975,9).
nees=e'*(P_out\e);                    %NEES = e'*inv(P)*e (con \ e' piu' stabile)
nees_band=[nees;2.7;19.0];            %NEES e limiti inferiore/superiore al 95%

== matlab function encelado/Altimetro ==
  data: p input size=3; R parameter; h_meas output size=1; sigma_h0 parameter size=3; k_h parameter
function h_meas=fcn(p,R,sigma_h0,k_h)
%Altimetro radar: misura la quota del lander sopra un terreno sferico liscio di raggio R. 
%Prende la posizione vera dal plant e restituisce la quota "sporcata" dal rumore del sensore. Il rumore cresce con la quota.
%Blocco senza stato: non serve nessun Unit Delay.
%Sample time del blocco: dt_alt (0.1 s).

%QUOTA VERA
%Distanza dal centro di Encelado meno il raggio. Il terreno e' una sfera, quindi la quota non dipende dalla direzione ma solo da norm(p).
h=norm(p(:))-R(1);                    %quota vera (scalare); (1) garantisce uno scalare anche se R arriva come vettore

%MISURA CON IL RUMORE
%Rumore gaussiano a media nulla con deviazione standard che cresce linearmente con la quota (radar meno preciso da lontano).
sigma_h=sigma_h0(1)+k_h(1)*max(h,0);  %sigma del rumore; max evita sigma<sigma_h0 se h<0 (sotto il suolo)
h_meas=h+sigma_h*randn;               %quota misuratasura(un solo numero)

== matlab function encelado/Camera ==
  data: p input size=3; R parameter; p_cam output size=3; sigma_c0 parameter size=3; k_c parameter
function p_cam=fcn(p,R,sigma_c0,k_c)
%Camera (navigazione relativa al terreno): fornisce un fix di posizione 3D
%"sporcato" da rumore gaussiano uguale sui tre assi, che cresce con la quota.
%Blocco senza stato. Sample time: dt_cam.
h=norm(p(:))-R(1);                    %quota vera
sigma_c=max(sigma_c0(1),k_c(1)*h);    %sigma del rumore: 1% della quota, minimo sigma_c0
p_cam=p(:)+sigma_c*randn(3,1);        %posizione misurata

== matlab function encelado/Giroscopio ==
  settings: updateMethod=DISCRETE
  data: bg input; bg_next output; w input; w_meas output; sigma_v parameter; sigma_u parameter; dt_imu parameter
function [bg_next,w_meas]=fcn(bg,w,sigma_v, sigma_u, dt_imu)
%Giroscopio: misura la velocita' angolare vera (assi corpo) con rumore
%bianco e bias con random walk. Bias tenuto dal Unit Delay esterno (IC=bg0).
eta_v=(sigma_v/sqrt(dt_imu))*randn(3,1);   %rumore bianco discreto
w_meas=w+bg+eta_v;                          %misura
bg_true=bg;                                 %bias vero usato in questa misura
bg_next=bg+sigma_u*sqrt(dt_imu)*randn(3,1); %random walk del bias

== matlab function encelado/Star Tracker ==
  settings: updateMethod=DISCRETE
  data: q input; q_st output; sigma_st parameter
function q_st=fcn(q,sigma_st)
%Star tracker: misura l'assetto con un piccolo errore di rotazione casuale.
%Blocco senza stato. Sample time: dt_st.
q=q(:)/norm(q);
dth=sigma_st*randn(3,1);                 %errore di rotazione [rad]
dq=[1;dth/2]; dq=dq/norm(dq);            %quaternione dell'errore
q_st=[dq(1)*q(1)-dq(2:4)'*q(2:4);
      dq(1)*q(2:4)+q(1)*dq(2:4)-cross(dq(2:4),q(2:4))];  %q_st=dq x q
q_st=q_st/norm(q_st); %random walk del bias

== matlab function encelado/Moltiplicative Extended Kalman Filter ==
  settings: updateMethod=DISCRETE
  data: xa input; Pa input; xa_next output; w_meas input; q_st input; t input; dt_imu parameter; Pa_next output; q_hat output; w_hat output; sig_att output; sigma_v parameter; sigma_u parameter; sigma_st parameter; N_st parameter
function [xa_next,Pa_next,q_hat,w_hat,sig_att]=fcn(xa,Pa,w_meas,q_st,t,dt_imu,sigma_v,sigma_u,sigma_st, N_st)
%Filtro d'assetto (MEKF): correzione con lo star tracker + previsione con il giroscopio.
%Stato: xa=[q_hat;bg_hat] (7x1), covarianza Pa 6x6 su [dtheta;dbg].

q_hat=xa(1:4)/norm(xa(1:4)); bg_hat=xa(5:7);
k=round(t/dt_imu);                    %numero del passo

%CORREZIONE CON LO STAR TRACKER
if mod(k,N_st)==0
    qi=[q_hat(1);-q_hat(2:4)];        %inverso di q_hat
    dqr=qm(q_st(:)/norm(q_st),qi);    %rotazione tra misura e stima
    if dqr(1)<0
        dqr=-dqr;                     %stesso assetto, emisfero positivo
    end
    y=2*dqr(2:4);                     %innovazione (angolo piccolo) 3x1
    H=[eye(3) zeros(3)];              %lo star tracker vede solo l'angolo
    Rs=sigma_st^2*eye(3);
    S=H*Pa*H'+Rs;                     %3x3
    K=Pa*H'/S;                        %guadagno 6x3
    dx=K*y;                           %correzione [dtheta;dbg]
    dq=[1;dx(1:3)/2];                 %piccola rotazione correttiva
    q_hat=qm(dq,q_hat);
    q_hat=q_hat/norm(q_hat);          %reset: l'errore passa dentro q_hat
    bg_hat=bg_hat+dx(4:6);
    IKH=eye(6)-K*H;
    Pa=IKH*Pa*IKH'+K*Rs*K';           %forma di Joseph
end

%USCITE AL PASSO k (dopo la correzione)
w_hat=w_meas-bg_hat;                  %velocita' angolare stimata
sig_att=sqrt(abs(diag(Pa)));          %sigma di [dtheta;dbg]

%PROPAGAZIONE DELL'ASSETTO
phi=w_hat*dt_imu;                     %rotazione nel passo [rad]
nphi=norm(phi);
if nphi>1e-12
    dq=[cos(nphi/2);sin(nphi/2)*phi/nphi];
else
    dq=[1;phi/2];
end
q_next=qm(dq,q_hat);
q_next=q_next/norm(q_next);
xa_next=[q_next;bg_hat];

%PROPAGAZIONE DELLA COVARIANZA
W=[0 -w_hat(3) w_hat(2);w_hat(3) 0 -w_hat(1);-w_hat(2) w_hat(1) 0];
F=[-W -eye(3);zeros(3,6)];
Phi=eye(6)+F*dt_imu+0.5*(F*F)*dt_imu^2;
Qd=blkdiag(sigma_v^2*dt_imu*eye(3),sigma_u^2*dt_imu*eye(3));
Pa_next=Phi*Pa*Phi'+Qd;
Pa_next=0.5*(Pa_next+Pa_next');

function r=qm(p,q)
%prodotto di quaternioni coerente con A(q): A(p x q)=A(p)A(q)
r=[p(1)*q(1)-p(2:4)'*q(2:4);
   p(1)*q(2:4)+q(1)*p(2:4)-cross(p(2:4),q(2:4))];

== matlab function encelado/MATLAB Function2 ==
  data: q input; eth_band output; q_hat input; sig_att input
function eth_band=fcn(q,q_hat,sig_att)
%Errore d'assetto: confronta l'assetto stimato dal MEKF con quello vero
%(noto solo in simulazione) per il test +-3sigma.
%L'errore e' la piccola rotazione dq che porta q_hat su q: q=dq x q_hat,
%stessa convenzione con cui il MEKF definisce dtheta nella covarianza Pa.
%q vero passato per Zero-Order Hold con dt_imu (stesso istante della stima).
%Blocco senza stato.

%QUATERNIONE D'ERRORE
q=q(:)/norm(q);                       %quaternione vero normalizzato
qi=[q_hat(1);-q_hat(2:4)];            %inverso (coniugato) di q_hat: vale perche' q_hat e' unitario
dq=[q(1)*qi(1)-q(2:4)'*qi(2:4);
    q(1)*qi(2:4)+qi(1)*q(2:4)-cross(q(2:4),qi(2:4))];  %dq=q x inv(q_hat), stesso prodotto di qm
if dq(1)<0
    dq=-dq;                           %q e -q sono lo stesso assetto: si sceglie dq vicino a [1;0;0;0]
end

%ANGOLO D'ERRORE E BANDA
%Per rotazioni piccole dq ~ [1;dtheta/2], quindi dtheta ~ 2*parte vettoriale.
dth=2*dq(2:4);                        %errore d'angolo sui tre assi [rad]
eth_band=[dth(1);3*sig_att(1);-3*sig_att(1)]; %errore attorno a x e banda: sig_att(1)=sigma di dtheta_x

== matlab function encelado/Position Dynamics Plant/Jacobi per verificare 3BP ==
  data: p input; C output; dp input; mu parameter; n parameter
function C = fcn(p,dp,mu, n)
x=p(1); y=p(2); z=p(3);
C=1/2*(norm(dp))^2 -3/2*n^2*x^2 +1/2*n^2*z^2 -mu/norm(p);

== matlab function encelado/Position Dynamics Plant/3BP ==
  data: ddx output size=1; T input; p input; dp input; ddy output size=1; ddz output size=1; n parameter; mu parameter; m input; kS parameter; kC parameter; kw parameter
function [ddx,ddy,ddz]= fcn(T,p,dp, n, mu, m, kS, kC, kw)
%p e dp entrano come colonna, ok
x=p(1); y=p(2); z=p(3);
dx=dp(1); dy=dp(2); %dz=dp(3);
Tx=T(1); Ty=T(2); Tz=T(3);
ddx= kC*2*n*dy +kw*n^2*x +kS*2*n^2*x -mu*x/(norm(p)^3) +Tx/m;
ddy=-kC*2*n*dx +kw*n^2*y -kS*n^2*y   -mu*y/(norm(p)^3) +Ty/m;
ddz=-kS*n^2*z                        -mu*z/(norm(p)^3) +Tz/m;

== matlab function encelado/Position Dynamics Plant/Tsiolkowsky ==
  data: T input; dm output; Isp parameter; g0 parameter
function dm=fcn(T,Isp, g0)
dm=-norm(T)/(Isp*g0);

== matlab function encelado/ZEM-ZEV-nl ==
  data: p input; T_des output; dp input; m input; n parameter; pf parameter; kC parameter; kS parameter; kw parameter; vf parameter; mu parameter; R parameter; tgo_min parameter; a_cmd output; Gam parameter; tgo output
function [T_des, a_cmd,tgo]=fcn(p,dp,m,n, pf, kC, kS, kw, vf, mu,R,tgo_min,Gam)
x=p(1); y=p(2); z=p(3);
dx=dp(1); dy=dp(2); dz=dp(3);
r=norm(p);
ddx= kC*2*n*dy +kw*n^2*x +kS*2*n^2*x -mu*x/r^3;
ddy=-kC*2*n*dx +kw*n^2*y -kS*n^2*y   -mu*y/r^3;
ddz=-kS*n^2*z                        -mu*z/r^3;
g=[ddx ddy ddz]';

%Newton per trovare il tgo della quartica
D=pf-p; v=dp; w=vf;
c4=Gam+0.5*(g'*g);
c2=-2*(v'*v+v'*w+w'*w);
c1=12*(D'*(v+w));
c0=-18*(D'*D);
f=@(t) c4*t^4+c2*t^2+c1*t+c0;
df=@(t) 4*c4*t^3+2*c2*t+c1;
t=1000;
for k=1:20
    t=t-f(t)/df(t);
end
tgo=max(t,tgo_min);
%Fine Newton

ZEM=pf-p-dp*tgo-0.5*g*tgo^2;
ZEV=vf-dp-g*tgo;
a_cmd=6*ZEM/tgo^2-2*ZEV/tgo;
T_des=m*a_cmd;




%ZEM ZEV "NORMALE"
% x=p(1); y=p(2); z=p(3);
% dx=dp(1); dy=dp(2); dz=dp(3);
% r=norm(p);
% ddx= kC*2*n*dy +kw*n^2*x +kS*2*n^2*x -mu*x/r^3;
% ddy=-kC*2*n*dx +kw*n^2*y -kS*n^2*y   -mu*y/r^3;
% ddz=-kS*n^2*z                        -mu*z/r^3;
% g=[ddx ddy ddz]';
% if t<tf
%     tgo=max(tf-t,10);
%     ZEM=pf-p-dp*tgo-0.5*g*tgo^2;
%     ZEV=vf-dp-g*tgo;
%     a_cmd=6*ZEM/tgo^2 -2*ZEV/tgo;
% else
%     u=p/r;
%     a_cmd=-g+(-1*u-dp)/10;
% end
% T_des=m*a_cmd;

== matlab function encelado/MATLAB Function ==
  data: p input; h output; dp input; v_ver output; v_hor output; R parameter
function [h,v_ver,v_hor]=fcn(p,dp,R)
u=p/norm(p);
h=norm(p)-R;
v_ver=dp'*u;
v_hor=norm(dp-v_ver*u);
